simulink model "manuel_pid_yedek"  (R2026a)
settings: Solver=VariableStepAuto
settings Model: Creator=seman  LastModifiedBy=seman

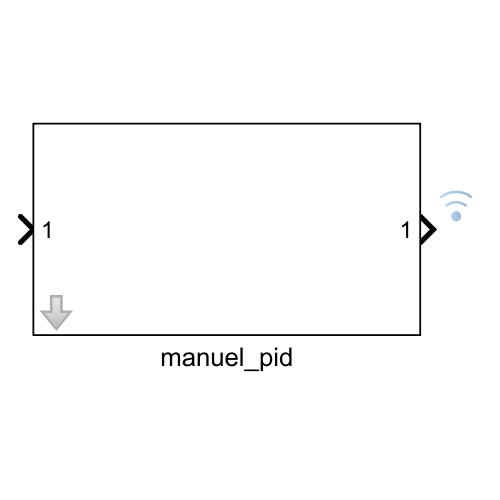
[thumbnail: Simulink's stored preview of the top-level diagram]
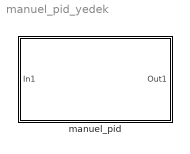
== system manuel_pid_yedek ==
  manuel_pid : Subsystem  mask{kp=175*0.6, ki=1.2*(175/0.33), kd=0.15*175*0.33}
      mask prompts: kp "proportional"
      mask DialogControl Container1 Prompt: Parameters

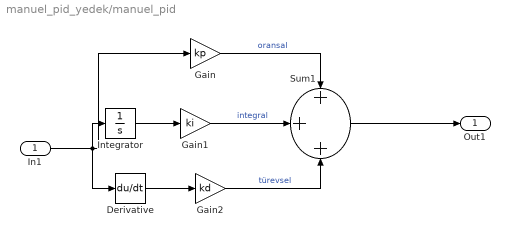
== system manuel_pid_yedek/manuel_pid ==
  In1 : Inport
  Derivative : Derivative
  Gain : Gain  Gain=kp
  Gain1 : Gain  Gain=ki
  Gain2 : Gain  Gain=kd
  Integrator : Integrator
  Sum1 : Sum  Inputs=+++
  Out1 : Outport
  wires:
  Derivative/1 -> Gain2/1
  Sum1/1 -> Out1/1
  Gain2/1 -> Sum1/3  "türevsel"
  In1/1 -> Derivative/1, Gain/1, Integrator/1
  Gain1/1 -> Sum1/2  "integral"
  Integrator/1 -> Gain1/1
  Gain/1 -> Sum1/1  "oransal"
